simulink model "L3_Predictor_Smith"  (R2025b)
settings: Solver=VariableStepAuto  StartTime=0.0  StopTime=20  RelTol=1e-3
values from neighbouring files (symbols this model uses):
  k_medie = 0.72245    [L2_PRELUCRARE_IDENTIFICARE.m]    (also in L3_Prelucrarea_Regulatorului_PI_PredictorSmith.m; L7_Prelucrare_identificare.m = 0.8195)
  Ki = Kp/Ti    (= 0.692089417953)    [L3_Prelucrarea_Regulatorului_PI_PredictorSmith.m]
  Kp = 1.3    [L3_DISCRETIZARE_PoliZerouri.m]    (also in L3_Prelucrarea_Regulatorului_PI_PredictorSmith.m = 1.51740604886)
  L_medie = 0.75    [L2_PRELUCRARE_IDENTIFICARE.m]    (also in L3_Prelucrarea_Regulatorului_PI_PredictorSmith.m; L7_Prelucrare_identificare.m = 1.8)
  T_medie = 2.1925    [L2_PRELUCRARE_IDENTIFICARE.m]    (also in L3_Prelucrarea_Regulatorului_PI_PredictorSmith.m; L7_Prelucrare_identificare.m = 3.1538)
libraries: slpidlib x1
settings Model: Creator=elisa  LastModifiedBy=elisa

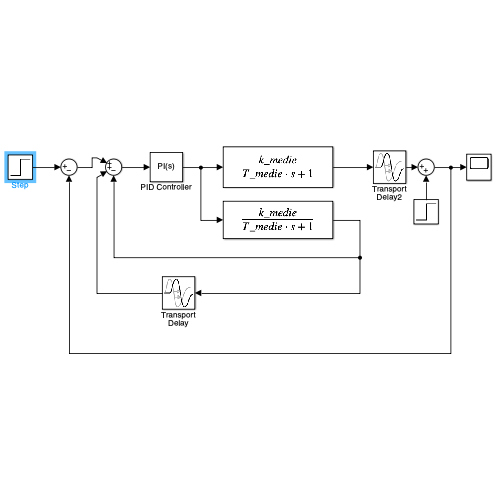
[thumbnail: Simulink's stored preview of the top-level diagram]
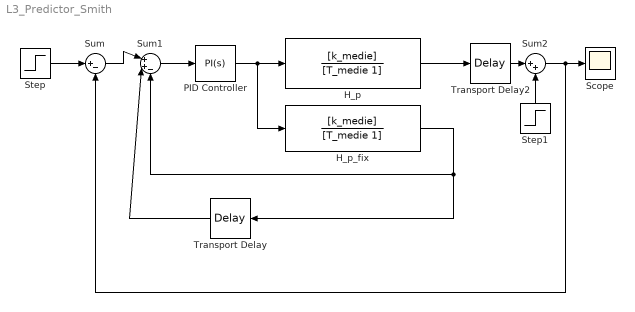
== system L3_Predictor_Smith ==
  H_p : TransferFcn  Numerator=[k_medie]  Denominator=[T_medie 1]
  H_p_fix : TransferFcn  Numerator=[k_medie]  Denominator=[T_medie 1]
  PID Controller : slpidlib/PID Controller  Controller=PI  Form=Parallel  TimeDomain=Continuous-time  UseExternalTs=off  SampleTime=-1  IntegratorMethod=Forward Euler  FilterMethod=Forward Euler  ControllerParametersSource=internal  P=Kp  I=Ki  UseKiTs=off  D=0  UseExternalDerivativeSource=off  N=100  UseFilter=on  TunerSelectOption=Transfer Function Based (PID Tuner App)  InitialConditionSource=internal  InitialConditionForIntegrator=0  InitialConditionForFilter=0  DifferentiatorICPrevScaledInput=0  ExternalReset=none  TrackingMode=off  Kt=1  LimitOutput=off  SatLimitsSource=internal  UpperSaturationLimit=inf  LowerSaturationLimit=-inf  LinearizeAsGain=on  AntiWindupMode=none  Kb=1  LimitIntegrator=off  UpperIntegratorSaturationLimit=inf  LowerIntegratorSaturationLimit=-inf  POutMin=[]  POutMax=[]  IOutMin=[]  IOutMax=[]  DOutMin=[]  DOutMax=[]  NOutMin=[]  NOutMax=[]  SumOutMin=[]  SumOutMax=[]  SaturationOutMin=[]  SaturationOutMax=[]  PParamMin=[]  PParamMax=[]  IParamMin=[]  IParamMax=[]  DParamMin=[]  DParamMax=[]  NParamMin=[]  NParamMax=[]  KbParamMin=[]  KbParamMax=[]  KtParamMin=[]  KtParamMax=[]  KbOutMin=[]  KbOutMax=[]  KtOutMin=[]  KtOutMax=[]  IntegratorOutMin=[]  IntegratorOutMax=[]  FilterOutMin=[]  FilterOutMax=[]  SumI1OutMin=[]  SumI1OutMax=[]  SumI2OutMin=[]  SumI2OutMax=[]  SumI3OutMin=[]  SumI3OutMax=[]  SumI4OutMin=[]  SumI4OutMax=[]  SumDOutMin=[]  SumDOutMax=[]  DifferentiatorOutMin=[]  DifferentiatorOutMax=[]  FilterDiffOutCoefMin=[]  FilterDiffOutCoefMax=[]  ReciprocalOutMin=[]  ReciprocalOutMax=[]  SumDenOutMin=[]  SumDenOutMax=[]  SumNumOutMin=[]  SumNumOutMax=[]  DivideOutMin=[]  DivideOutMax=[]  UdiffTsProdOutMin=[]  UdiffTsProdOutMax=[]  NTsProdOutMin=[]  NTsProdOutMax=[]  UintegralTsProdOutMin=[]  UintegralTsProdOutMax=[]  UngainTsProdOutMin=[]  UngainTsProdOutMax=[]  ClampingZeroOutDataTypeStr=Inherit: Inherit via back propagation  ClampingZeroOutMin=[]  ClampingZeroOutMax=[]  FilterDenConstantOutDataTypeStr=Inherit: Inherit via back propagation  FilterDenConstantOutMin=[]  FilterDenConstantOutMax=[]  PCopyOutDataTypeStr=Inherit: Inherit via back propagation  PCopyOutMin=[]  PCopyOutMax=[]  NCopyOutDataTypeStr=Inherit: Inherit via back propagation  NCopyOutMin=[]  NCopyOutMax=[]  IntegratorContinuousStateAttributes=''  IntegratorStateMustResolveToSignalObject=off  IntegratorRTWStateStorageClass=Auto  FilterContinuousStateAttributes=''  FilterStateMustResolveToSignalObject=off  FilterRTWStateStorageClass=Auto  ParallelPVariant=InternalParameters  IdealPVariant=Disabled  IVariant=InternalParameters  DVariant=Disabled  IntegratorVariant=Continuous  SatVariant=Disabled  AWVariant=Passthrough  PCopyVariant=Disabled  TRVariant=Disabled  FdbkBlocksVariant=Forward  IdealPFdbkVariant=Disabled  SatFdbkVariant=Disabled  DerivativeFilterVariant=Disabled  NVariant=Disabled  NCopyVariant=Disabled_SignalSpec  FilterICVariant=Disabled  IntegratorICVariant=InternalICs  ExternalResetVariant=Disabled  TRSumVariant=Passthrough  SumFdbkVariant=Disabled  SumVariant=Sum_PI  TsampFilterVariant=InternalTs  TsampNgainVariant=Passthrough  TsampIntegralVariant=Disabled_SignalSpec  ExternalSaturationOutDataTypeStr=Inherit: Same as second input  DerivativeSourceVariant=Disabled  PreIntVariant=InternalPreInt
  Scope : Scope
      settings: ActiveDisplayYMinimum=-2.4991715568074309  ActiveDisplayYMaximum=122.49254401126692
  Step : Step  Time=0  After=110  SampleTime=0
  Step1 : Step  Time=0  After=10  SampleTime=0
  Sum : Sum  Inputs=|+-
  Sum1 : Sum  Inputs=|++-
  Sum2 : Sum  Inputs=|++
  Transport Delay : TransportDelay  DelayTime=L_medie
  Transport Delay2 : TransportDelay  DelayTime=L_medie
  wires:
  Sum1/1 -> PID Controller/1
  Sum/1 -> Sum1/1
  Step/1 -> Sum/1
  PID Controller/1 -> H_p_fix/1, H_p/1
  H_p_fix/1 -> Sum1/3, Transport Delay/1
  Transport Delay/1 -> Sum1/2
  Sum2/1 -> Sum/2, Scope/1
  Step1/1 -> Sum2/2
  H_p/1 -> Transport Delay2/1
  Transport Delay2/1 -> Sum2/1
